simulink model "AXU5EV_Hybrid_ClosedLoop"  (R2026b)
settings: Solver=FixedStepDiscrete  StopTime=6  FixedStep=Ts_Plant
InitFcn:
  | m1a_require_float_init(bdroot);
undefined symbols (not defined in the file): Alignment_Enable, AX01B_Use_C, AX01B_Use_RTL, DiscIntNeverNeededParam, Host_Close_Loop_EN, Host_Id_A, Host_Iq_A, Host_Iq_Test_Mode, Host_Move_Request, Host_PI_Reset_EN, Host_Position_Loop_EN, Host_PWM_EN, Host_Replay_EN, Host_Speed_mmps, Host_Target_mm, Init_Reset, Init_Start, M1A_PWM_Update_Delay_s, PMLSM_Bv_N_per_mps, PMLSM_deadtime_current_eps_A, PMLSM_deadtime_ratio, PMLSM_Fc_N, PMLSM_Kf_peak_N_per_Apeak, PMLSM_Ld_H, PMLSM_Lq_H, PMLSM_M_kg, PMLSM_psi_f_Wb, PMLSM_Rs_ohm, PMLSM_tau_NN_m, PMLSM_theta_offset_rad, PMLSM_Ts_s, PMLSM_v_eps_mps, Simulation_Travel_Fault, Tau_e_mm, theta_align_const, Theta_Offset_Fine, Ts_ACR, Ts_Plant
settings Model: Creator=lww  LastModifiedBy=lww
settings DataIOCC: SaveOutput=off  SaveTime=off

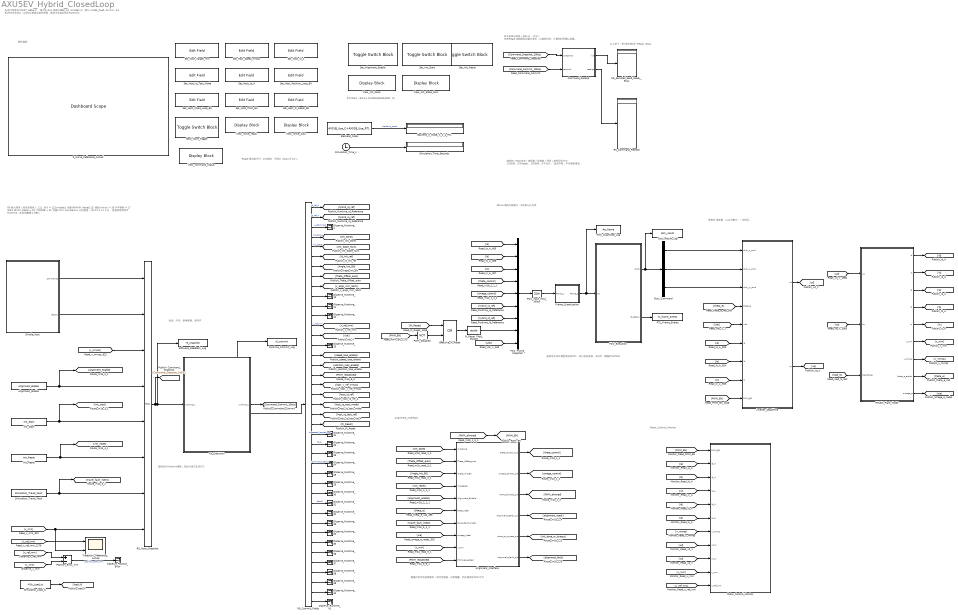
== system AXU5EV_Hybrid_ClosedLoop ==
  note: ​
      | 选择运行Runtime模型，或运行由它生成的C
  note: ​
      | 选择定点FOC模型或实际RTL，执行坐标变换、电流PI、限幅和SVPWM
  note: Alignment_Interface
  note: 根据对齐状态选择固定／实时控制角、应用偏置，并处理实际PWM许可
  note: 轨迹、外环、参考管理、原对齐
  note: Motor_Control_Monitor
  note: 操作面板
  note: 原电机/逆变器，1 µs对象步；一次死区。
  note: 100 µs调用与帧提交；共同50 µs应用
  note: 手动Start；原0.5 A及10000/30000/2000拍
  note: Ready是当拍许可；0时拒绝、不排队（Busy可为0）。
  note: R5 输入顺序（按当前接线）
      | 1:11 命令 → 12:14 replay[速度/PWM/PI_Reset]
      | 15 速度(mm/s) → 16 对齐使能 → 17 Start
      | 18 Init_Reset → 19 行程故障 → 20 位置(mm)
      | Mux/Demux 分组宽度：[11 3 1 1 1 1 1 1]
      | 改变顺序须同步 Runtime，并显式重建 C MEX。
  note: 先运行同目录 START_HERE.m，再点击 Run
      | 参数只编辑 init_AXU5EV.m；默认 model_fixed / 10 mm / 5 s
      | Runtime生成C；Control是独立组件来源，修改不会自动同步Runtime。
  note: 命令采样与回执（100 us，只读）
      | 左侧Ready会随原到位窗口变化；以接收时间、计数和段号确认结果。
  note: 从上到下：R5采样Send / Ready / Busy
  note: 接收秒 / Host状态 / 接受数 / 拒绝数 / 段号 / 接受目标mm
      | 2已接受，3未Ready，5同目标，6不允许；7运动中断，不代表新请求。
  Alignment_Enable : Constant  Value=Alignment_Enable  OutDataTypeStr=double  SampleTime=Ts_ACR
  Alignment_Interface : Subsystem
  Backend_0_Model_1_C_2_RTL : Display
  Backend_Code : Constant  Value=AX01B_Use_C+AX01B_Use_RTL
  Command_Receipt : Subsystem
  Duty_Command : Demux  Outputs=3
  Duty_Result_Log : ToWorkspace  VariableName=duty_result  SaveFormat=Timeseries  SampleTime=Ts_ACR
  Effective_PI_Reset : Logic  Operator=OR  AllPortsSameDT=off  OutDataTypeStr=boolean
  FOC_Execution : Subsystem  Variant=on
  FOC_Frame_Snapshot : Mux  Inputs=9
  FOC_Input_Hold_100us : ZeroOrderHold  SampleTime=Ts_ACR
  FOC_Quantized_Log : ToWorkspace  VariableName=foc_frame  SaveFormat=Timeseries  SampleTime=Ts_ACR
  Frame_Quantization : Subsystem
  Init_Reset : Constant  Value=Init_Reset  SampleTime=Ts_ACR
  Init_Start : Constant  Value=Init_Start  SampleTime=Ts_ACR
  Inverter_DeadTime : Subsystem
  Motor_Control_Monitor : Subsystem
  Observe_Position_Error : Terminator
  Observe_Runtime_{3,10..12,15,24..41} (23 alike) : Terminator
  PI_Reset_Field_Double : DataTypeConversion  OutDataTypeStr=double  SaturateOnIntegerOverflow=off  RndMeth=Floor
  PMLSM_Plant_Model : Subsystem
  PWM_Disabled : Logic  Operator=NOT  AllPortsSameDT=off  OutDataTypeStr=boolean
  Position_Error_mm : Sum  Inputs=+-
  R5_Command_Receipt : Display
  R5_Commit_Fields : Demux  Description=runtime_y（41字段）：1:3 id/iq/v参考；4:12 对齐；13 x_ref_mm；14:23 运行字段；24 接受目标；25 Busy；27 status；31 Ready；32:36 计数/段/中断；37:41 轨迹配置。详见同目录运行说明。  Outputs=41
  R5_Execution : Subsystem  Variant=on
  R5_Input_Snapshot : Mux  Description=runtime_u（20字段）：命令[1:11]，replay[12:14]，v_mmps[15]，Alignment_Enable[16]，Init_Start[17]，Init_Reset[18]，travel_fault[19]，x_mm[20]。保持当前接线顺序，Runtime Demux必须同步。  Inputs=[11 3 1 1 1 1 1 1]
  R5_Sampled_Send_Ready_Busy : Display
  RTL_Frame_Events : ToWorkspace  VariableName=rtl_frame_events  SaveFormat=Timeseries  SampleTime=-1
  Runtime_Commit_Log : ToWorkspace  VariableName=r5_commit  SaveFormat=Timeseries  SampleTime=Ts_ACR
  S_Curve_Reference_Actual : DashboardScope  FontColor=[0.0, 0.0, 0.0]
  Send_Move_Toggle : ToggleSwitchBlock
  Set_Alignment_Enable : ToggleSwitchBlock
  Set_Host_Close_Loop_EN : EditField  ShowInitialText=on  Alignment=Center
  Set_Host_Id_A : EditField  ShowInitialText=on  Alignment=Center
  Set_Host_Iq_A : EditField  ShowInitialText=on  Alignment=Center
  Set_Host_Iq_Test_Mode : EditField  ShowInitialText=on  Alignment=Center
  Set_Host_PI_Reset_EN : EditField  ShowInitialText=on  Alignment=Center
  Set_Host_PWM_EN : EditField  ShowInitialText=on  Alignment=Center
  Set_Host_Position_Loop_EN : EditField  ShowInitialText=on  Alignment=Center
  Set_Host_Speed_mmps : EditField  ShowInitialText=on  Alignment=Center
  Set_Host_Target_mm : EditField  ShowInitialText=on  Alignment=Center
  Set_Init_Reset : ToggleSwitchBlock
  Set_Init_Start : ToggleSwitchBlock
  Simple_Host : Subsystem
  Simulation_Load_N : FromWorkspace  VariableName=M1A_Load_ts  SampleTime=Ts_Plant  Interpolate=off  OutputAfterFinalValue=Holding final value
  Simulation_Time_Seconds : Display
  Simulation_Time_s : Clock
  Simulation_Travel_Fault : Constant  Value=Simulation_Travel_Fault  OutDataTypeStr=double  SampleTime=Ts_ACR
  Software_Feedback_Log : ToWorkspace  VariableName=r5_snapshot  SaveFormat=Timeseries  SampleTime=Ts_ACR
  Trajectory_Reference_Actual : Scope  NumInputPorts=2
      settings: ActiveDisplayYMinimum=0.99182264665726316  ActiveDisplayYMaximum=1.0007838303678565
  View_Init_Done : DisplayBlock  Transparency=1  GridColor=[0.502, 0.502, 0.502]
  View_Init_State_Num : DisplayBlock  Transparency=1  GridColor=[0.502, 0.502, 0.502]
  View_command_status : DisplayBlock  Transparency=1  GridColor=[0.502, 0.502, 0.502]
  View_move_busy : DisplayBlock  Transparency=1  GridColor=[0.502, 0.502, 0.502]
  View_move_ready : DisplayBlock  Transparency=1  GridColor=[0.502, 0.502, 0.502]
  wires:
  [PWM_EN] -> PWM_Disabled/1
  PMLSM_Plant_Model/6(x_mm) -> [x_mm]
  PMLSM_Plant_Model/7(v_mmps) -> [v_mmps]
  PMLSM_Plant_Model/3(ia) -> [ia]
  PMLSM_Plant_Model/4(ib) -> [ib]
  PMLSM_Plant_Model/5(ic) -> [ic]
  PMLSM_Plant_Model/8(theta_e_actual) -> [theta_e]
  PMLSM_Plant_Model/9(omega_e) -> [we]
  PMLSM_Plant_Model/1(id) -> [id]
  PMLSM_Plant_Model/2(iq) -> [iq]
  [load_N] -> PMLSM_Plant_Model/3(load_force)
  [uq] -> PMLSM_Plant_Model/2(vq)
  [ud] -> PMLSM_Plant_Model/1(vd)
  Simulation_Load_N/1 -> [load_N]
  [theta_e] -> Alignment_Interface/6(theta_ideal)
  [we] -> Alignment_Interface/8(omega_ideal)
  Alignment_Interface/1(theta_control_out) -> [theta_control]
  Alignment_Interface/2(omega_control_out) -> [omega_control]
  Alignment_Interface/3(PWM_allowed_out) -> [PWM_allowed]
  [PWM_allowed] -> [PWM_EN]
  Alignment_Interface/4(alignment_ready_out) -> [alignment_ready]
  Alignment_Interface/5(done_or_bypass_out) -> [init_done_or_bypass]
  Alignment_Interface/6(alignment_fault_out) -> [alignment_fault]
  [alignment_enable] -> Alignment_Interface/5(Alignment_Enable)
  [init_reset] -> Alignment_Interface/4(Init_Reset)
  [travel_fault_inject] -> Alignment_Interface/7(travel_fault_inject)
  [PWM_requested] -> Alignment_Interface/10(PWM_requested)
  [Init_Done] -> Alignment_Interface/1(Init_Done)
  [Angle_Init_EN] -> Alignment_Interface/3(Angle_Init_EN)
  [Theta_Offset_auto] -> Alignment_Interface/2(Theta_Offset_auto)
  [x_mm] -> Alignment_Interface/9(x_mm)
  [omega_control] -> FOC_Frame_Snapshot/5
  [theta_control] -> FOC_Frame_Snapshot/4
  [ic] -> FOC_Frame_Snapshot/3
  [ib] -> FOC_Frame_Snapshot/2
  [ia] -> FOC_Frame_Snapshot/1
  [PI_Reset] -> Effective_PI_Reset/1
  PWM_Disabled/1 -> Effective_PI_Reset/2
  FOC_Frame_Snapshot/1 -> FOC_Input_Hold_100us/1
  PI_Reset_Field_Double/1 -> FOC_Frame_Snapshot/8
  Effective_PI_Reset/1 -> PI_Reset_Field_Double/1
  [ic] -> Inverter_DeadTime/8(ic)
  [ib] -> Inverter_DeadTime/7(ib)
  [ia] -> Inverter_DeadTime/6(ia)
  [theta_e] -> Inverter_DeadTime/4(theta_e)
  Inverter_DeadTime/1(vd) -> [ud]
  Inverter_DeadTime/2(vq) -> [uq]
  [PWM_EN] -> Inverter_DeadTime/9(PWM_EN)
  [x_ref_mm] -> Motor_Control_Monitor/11(x_ref_mm)
  [x_mm] -> Motor_Control_Monitor/10(x_mm)
  [uq] -> Motor_Control_Monitor/9(vq_V)
  [ud] -> Motor_Control_Monitor/8(vd_V)
  [v_mmps] -> Motor_Control_Monitor/7(v_mmps)
  [iq] -> Motor_Control_Monitor/6(iq_A)
  [id] -> Motor_Control_Monitor/5(id_A)
  [ic] -> Motor_Control_Monitor/4(ic_A)
  [ib] -> Motor_Control_Monitor/3(ib_A)
  [ia] -> Motor_Control_Monitor/2(ia_A)
  [PWM_EN] -> Motor_Control_Monitor/1(PWM_EN)
  Duty_Command/3 -> Inverter_DeadTime/3(duty_w_cmd)
  Duty_Command/2 -> Inverter_DeadTime/2(duty_v_cmd)
  Duty_Command/1 -> Inverter_DeadTime/1(duty_u_cmd)
  FOC_Execution/1(Out1) -> Duty_Result_Log/1, Duty_Command/1
  FOC_Execution/2(rtl_status) -> RTL_Frame_Events/1
  R5_Commit_Fields/3 -> Observe_Runtime_3/1  "v_ref_mmps"
  R5_Commit_Fields/10 -> Observe_Runtime_10/1
  R5_Commit_Fields/11 -> Observe_Runtime_11/1
  R5_Commit_Fields/12 -> Observe_Runtime_12/1
  R5_Commit_Fields/15 -> Observe_Runtime_15/1
  R5_Commit_Fields/24 -> Observe_Runtime_24/1  "accepted_target_mm"
  R5_Commit_Fields/25 -> Observe_Runtime_25/1  "Busy"
  R5_Commit_Fields/26 -> Observe_Runtime_26/1
  R5_Commit_Fields/27 -> Observe_Runtime_27/1  "command_status"
  R5_Commit_Fields/28 -> Observe_Runtime_28/1
  R5_Commit_Fields/29 -> Observe_Runtime_29/1
  R5_Commit_Fields/30 -> Observe_Runtime_30/1
  R5_Commit_Fields/31 -> Observe_Runtime_31/1  "Ready"
  R5_Commit_Fields/32 -> Observe_Runtime_32/1
  R5_Commit_Fields/33 -> Observe_Runtime_33/1
  R5_Commit_Fields/34 -> Observe_Runtime_34/1
  R5_Commit_Fields/35 -> Observe_Runtime_35/1
  R5_Commit_Fields/36 -> Observe_Runtime_36/1
  R5_Commit_Fields/37 -> Observe_Runtime_37/1
  R5_Commit_Fields/38 -> Observe_Runtime_38/1
  R5_Commit_Fields/39 -> Observe_Runtime_39/1
  R5_Commit_Fields/40 -> Observe_Runtime_40/1
  R5_Commit_Fields/41 -> Observe_Runtime_41/1
  R5_Commit_Fields/4 -> [Init_Done]  "Init_Done"
  R5_Commit_Fields/5 -> [Init_State_Num]  "Init_State"
  R5_Commit_Fields/6 -> [id_init_ref]
  R5_Commit_Fields/7 -> [Angle_Init_EN]
  R5_Commit_Fields/8 -> [Theta_Offset_auto]
  R5_Commit_Fields/9 -> [x_align_mm_latch]
  R5_Commit_Fields/13 -> [x_ref_mm]  "x_ref_mm"
  R5_Commit_Fields/16 -> [speed_loop_enable]
  R5_Commit_Fields/17 -> [position_loop_enable]
  R5_Commit_Fields/20 -> [host_id_ref]
  R5_Commit_Fields/21 -> [host_iq_test_mode]
  R5_Commit_Fields/22 -> [host_iq_test_ref]
  R5_Commit_Fields/19 -> [host_v_ref_mmps]
  R5_Commit_Fields/18 -> [PWM_requested]
  R5_Commit_Fields/23 -> [PI_Reset]
  FOC_Input_Hold_100us/1 -> Frame_Quantization/1(frame_u)
  Frame_Quantization/1(frame_q) -> FOC_Quantized_Log/1, FOC_Execution/1(In1)
  Alignment_Enable/1 -> [alignment_enable], R5_Input_Snapshot/4
  Init_Start/1 -> [init_start], R5_Input_Snapshot/5
  Init_Reset/1 -> [init_reset], R5_Input_Snapshot/6
  Simulation_Travel_Fault/1 -> [travel_fault_inject], R5_Input_Snapshot/7
  [x_ref_mm] -> Trajectory_Reference_Actual/1
  [x_mm] -> Trajectory_Reference_Actual/2, R5_Input_Snapshot/8
  Simple_Host/1(commands) -> R5_Input_Snapshot/1
  [v_mmps] -> R5_Input_Snapshot/3
  [hybrid_iq_ref] -> FOC_Frame_Snapshot/6
  [hybrid_id_ref] -> FOC_Frame_Snapshot/7
  R5_Commit_Fields/1 -> [hybrid_id_ref]  "id_ref_A"
  R5_Commit_Fields/2 -> [hybrid_iq_ref]  "iq_ref_A"
  R5_Commit_Fields/14 -> [Udc]
  [Udc] -> FOC_Frame_Snapshot/9
  Simple_Host/2(replay) -> R5_Input_Snapshot/2
  [Udc] -> Inverter_DeadTime/5(vdc)
  Position_Error_mm/1 -> Observe_Position_Error/1  "position_error_mm"
  [x_mm] -> Position_Error_mm/2
  [x_ref_mm] -> Position_Error_mm/1
  Simulation_Time_s/1 -> Simulation_Time_Seconds/1
  Backend_Code/1 -> Backend_0_Model_1_C_2_RTL/1  "backend_code"
  Command_Receipt/2(receipt) -> R5_Command_Receipt/1
  Command_Receipt/1(live) -> R5_Sampled_Send_Ready_Busy/1
  [Command_Commit_100us] -> Command_Receipt/2(commit)
  [Command_Snapshot_100us] -> Command_Receipt/1(snapshot)
  R5_Input_Snapshot/1 -> R5_Execution/1(runtime_u), Software_Feedback_Log/1, [Command_Snapshot_100us]
  R5_Execution/1(runtime_y) -> [Command_Commit_100us], Runtime_Commit_Log/1, R5_Commit_Fields/1

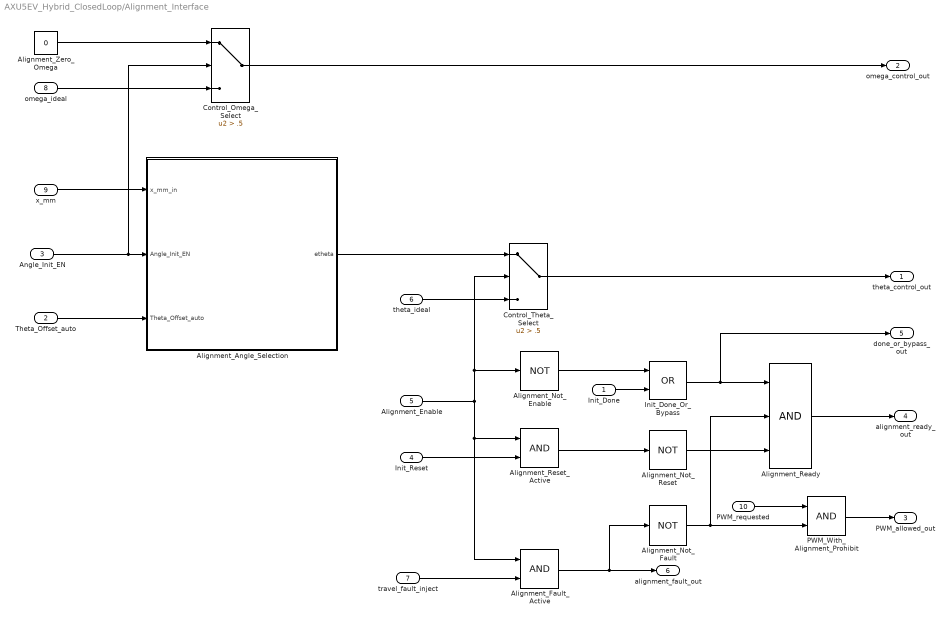
== system AXU5EV_Hybrid_ClosedLoop/Alignment_Interface ==
  Init_Done : Inport
  Theta_Offset_auto : Inport  Port=2
  Angle_Init_EN : Inport  Port=3
  Init_Reset : Inport  Port=4
  Alignment_Enable : Inport  Port=5
  theta_ideal : Inport  Port=6
  travel_fault_inject : Inport  Port=7
  omega_ideal : Inport  Port=8
  x_mm : Inport  Port=9
  PWM_requested : Inport  Port=10
  Alignment_Angle_Selection : Subsystem
  Alignment_Fault_Active : Logic  AllPortsSameDT=off  OutDataTypeStr=boolean
  Alignment_Not_Enable : Logic  Operator=NOT  AllPortsSameDT=off  OutDataTypeStr=boolean
  Alignment_Not_Fault : Logic  Operator=NOT  AllPortsSameDT=off  OutDataTypeStr=boolean
  Alignment_Not_Reset : Logic  Operator=NOT  AllPortsSameDT=off  OutDataTypeStr=boolean
  Alignment_Ready : Logic  Inputs=3  AllPortsSameDT=off  OutDataTypeStr=boolean
  Alignment_Reset_Active : Logic  AllPortsSameDT=off  OutDataTypeStr=boolean
  Alignment_Zero_Omega : Constant  Value=0
  Control_Omega_Select : Switch  Criteria=u2 > Threshold  Threshold=.5
  Control_Theta_Select : Switch  Criteria=u2 > Threshold  Threshold=.5
  Init_Done_Or_Bypass : Logic  Operator=OR  AllPortsSameDT=off  OutDataTypeStr=boolean
  PWM_With_Alignment_Prohibit : Logic  AllPortsSameDT=off  OutDataTypeStr=boolean
  theta_control_out : Outport
  omega_control_out : Outport  Port=2
  PWM_allowed_out : Outport  Port=3
  alignment_ready_out : Outport  Port=4
  done_or_bypass_out : Outport  Port=5
  alignment_fault_out : Outport  Port=6
  wires:
  Alignment_Zero_Omega/1 -> Control_Omega_Select/1
  travel_fault_inject/1 -> Alignment_Fault_Active/2
  x_mm/1 -> Alignment_Angle_Selection/1(x_mm_in)
  Alignment_Enable/1 -> Alignment_Fault_Active/1, Alignment_Reset_Active/1, Alignment_Not_Enable/1, Control_Theta_Select/2
  PWM_requested/1 -> PWM_With_Alignment_Prohibit/1
  omega_ideal/1 -> Control_Omega_Select/3
  theta_ideal/1 -> Control_Theta_Select/3
  Angle_Init_EN/1 -> Control_Omega_Select/2, Alignment_Angle_Selection/2(Angle_Init_EN)
  Init_Reset/1 -> Alignment_Reset_Active/2
  Theta_Offset_auto/1 -> Alignment_Angle_Selection/3(Theta_Offset_auto)
  Control_Omega_Select/1 -> omega_control_out/1
  Alignment_Angle_Selection/1(etheta) -> Control_Theta_Select/1
  PWM_With_Alignment_Prohibit/1 -> PWM_allowed_out/1
  Init_Done_Or_Bypass/1 -> done_or_bypass_out/1, Alignment_Ready/1
  Control_Theta_Select/1 -> theta_control_out/1
  Alignment_Fault_Active/1 -> Alignment_Not_Fault/1, alignment_fault_out/1
  Alignment_Not_Enable/1 -> Init_Done_Or_Bypass/1
  Alignment_Not_Reset/1 -> Alignment_Ready/3
  Alignment_Reset_Active/1 -> Alignment_Not_Reset/1
  Alignment_Not_Fault/1 -> Alignment_Ready/2, PWM_With_Alignment_Prohibit/2
  Alignment_Ready/1 -> alignment_ready_out/1
  Init_Done/1 -> Init_Done_Or_Bypass/2

== system AXU5EV_Hybrid_ClosedLoop/Command_Receipt ==
  snapshot : Inport
  commit : Inport  Port=2
  Receipt_Fields : MATLAB Function  TreatAsAtomicUnit=on
  Snapshot_100us : ZeroOrderHold  SampleTime=Ts_ACR
  live : Outport
  receipt : Outport  Port=2
  wires:
  Snapshot_100us/1 -> Receipt_Fields/1(snapshot)
  snapshot/1 -> Snapshot_100us/1
  commit/1 -> Receipt_Fields/2(commit)
  Receipt_Fields/1(live) -> live/1
  Receipt_Fields/2(receipt) -> receipt/1

== system AXU5EV_Hybrid_ClosedLoop/FOC_Execution ==
  note: 1) Add Subsystem or Model blocks as valid variant choices.
      | 2) You cannot connect blocks at this level. At simulation, connectivity is automatically
      | determined, based on the active variant and port name matching.
  In1 : Inport
  Fixed_Reference : Subsystem  VariantControl=AX01B_Use_RTL == 0
  P3_RTL : Subsystem  VariantControl=AX01B_Use_RTL == 1
  Out1 : Outport
  rtl_status : Outport  Port=2

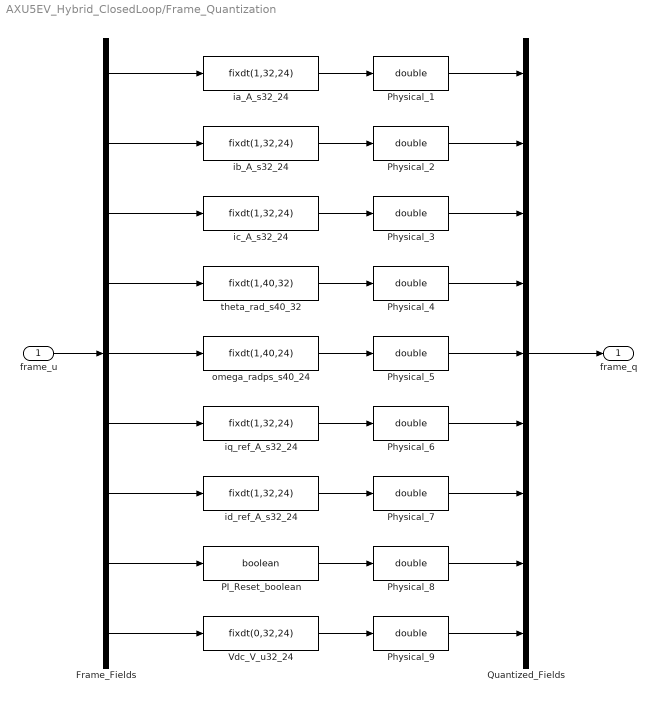
== system AXU5EV_Hybrid_ClosedLoop/Frame_Quantization ==
  frame_u : Inport
  Frame_Fields : Demux  Outputs=9
  PI_Reset_boolean : DataTypeConversion  OutDataTypeStr=boolean  RndMeth=Convergent
  Physical_{1..9} (9 alike) : DataTypeConversion  OutDataTypeStr=double  SaturateOnIntegerOverflow=off  RndMeth=Floor
  Quantized_Fields : Mux  Inputs=9
  Vdc_V_u32_24 : DataTypeConversion  OutDataTypeStr=fixdt(0,32,24)  RndMeth=Convergent
  ia_A_s32_24 : DataTypeConversion  OutDataTypeStr=fixdt(1,32,24)  RndMeth=Convergent
  ib_A_s32_24 : DataTypeConversion  OutDataTypeStr=fixdt(1,32,24)  RndMeth=Convergent
  ic_A_s32_24 : DataTypeConversion  OutDataTypeStr=fixdt(1,32,24)  RndMeth=Convergent
  id_ref_A_s32_24 : DataTypeConversion  OutDataTypeStr=fixdt(1,32,24)  RndMeth=Convergent
  iq_ref_A_s32_24 : DataTypeConversion  OutDataTypeStr=fixdt(1,32,24)  RndMeth=Convergent
  omega_radps_s40_24 : DataTypeConversion  OutDataTypeStr=fixdt(1,40,24)  RndMeth=Convergent
  theta_rad_s40_32 : DataTypeConversion  OutDataTypeStr=fixdt(1,40,32)  RndMeth=Convergent
  frame_q : Outport
  wires:
  Quantized_Fields/1 -> frame_q/1
  Physical_9/1 -> Quantized_Fields/9
  Vdc_V_u32_24/1 -> Physical_9/1
  Frame_Fields/9 -> Vdc_V_u32_24/1
  Physical_8/1 -> Quantized_Fields/8
  PI_Reset_boolean/1 -> Physical_8/1
  Frame_Fields/8 -> PI_Reset_boolean/1
  Physical_7/1 -> Quantized_Fields/7
  id_ref_A_s32_24/1 -> Physical_7/1
  Frame_Fields/7 -> id_ref_A_s32_24/1
  Physical_6/1 -> Quantized_Fields/6
  iq_ref_A_s32_24/1 -> Physical_6/1
  Frame_Fields/6 -> iq_ref_A_s32_24/1
  Physical_5/1 -> Quantized_Fields/5
  omega_radps_s40_24/1 -> Physical_5/1
  Frame_Fields/5 -> omega_radps_s40_24/1
  Physical_4/1 -> Quantized_Fields/4
  theta_rad_s40_32/1 -> Physical_4/1
  Frame_Fields/4 -> theta_rad_s40_32/1
  Physical_3/1 -> Quantized_Fields/3
  ic_A_s32_24/1 -> Physical_3/1
  Frame_Fields/3 -> ic_A_s32_24/1
  Physical_2/1 -> Quantized_Fields/2
  ib_A_s32_24/1 -> Physical_2/1
  Frame_Fields/2 -> ib_A_s32_24/1
  Physical_1/1 -> Quantized_Fields/1
  ia_A_s32_24/1 -> Physical_1/1
  Frame_Fields/1 -> ia_A_s32_24/1
  frame_u/1 -> Frame_Fields/1

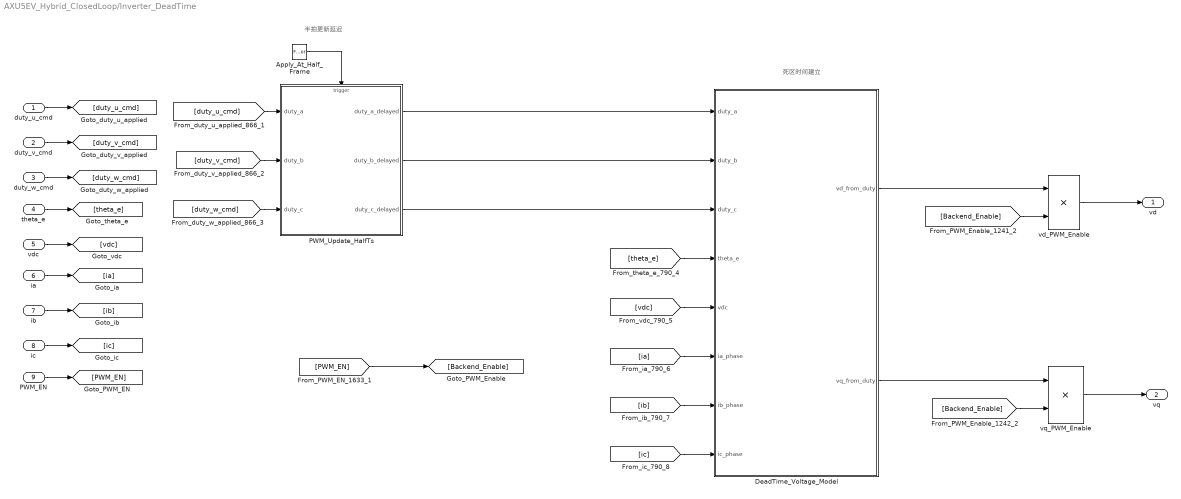
== system AXU5EV_Hybrid_ClosedLoop/Inverter_DeadTime ==
  note: 死区时间建立
  note: 半拍更新延迟
  duty_u_cmd : Inport
  duty_v_cmd : Inport  Port=2
  duty_w_cmd : Inport  Port=3
  theta_e : Inport  Port=4
  vdc : Inport  Port=5
  ia : Inport  Port=6
  ib : Inport  Port=7
  ic : Inport  Port=8
  PWM_EN : Inport  Port=9
  Apply_At_Half_Frame : FunctionCallGenerator  SampleTime=[Ts_ACR M1A_PWM_Update_Delay_s]
  DeadTime_Voltage_Model : Subsystem
  PWM_Update_HalfTs : Subsystem
  vd_PWM_Enable : Product  Inputs=**
  vq_PWM_Enable : Product  Inputs=**
  vd : Outport
  vq : Outport  Port=2
  wires:
  [PWM_EN] -> [Backend_Enable]
  [ic] -> DeadTime_Voltage_Model/8(ic_phase)
  [ib] -> DeadTime_Voltage_Model/7(ib_phase)
  [ia] -> DeadTime_Voltage_Model/6(ia_phase)
  [vdc] -> DeadTime_Voltage_Model/5(vdc)
  [theta_e] -> DeadTime_Voltage_Model/4(theta_e)
  [duty_w_cmd] -> PWM_Update_HalfTs/3(duty_c)
  [duty_v_cmd] -> PWM_Update_HalfTs/2(duty_b)
  [duty_u_cmd] -> PWM_Update_HalfTs/1(duty_a)
  PWM_EN/1 -> [PWM_EN]
  PWM_Update_HalfTs/3(duty_c_delayed) -> DeadTime_Voltage_Model/3(duty_c)
  PWM_Update_HalfTs/2(duty_b_delayed) -> DeadTime_Voltage_Model/2(duty_b)
  PWM_Update_HalfTs/1(duty_a_delayed) -> DeadTime_Voltage_Model/1(duty_a)
  ic/1 -> [ic]
  ib/1 -> [ib]
  ia/1 -> [ia]
  vdc/1 -> [vdc]
  theta_e/1 -> [theta_e]
  duty_u_cmd/1 -> [duty_u_cmd]
  duty_v_cmd/1 -> [duty_v_cmd]
  duty_w_cmd/1 -> [duty_w_cmd]
  [Backend_Enable] -> vd_PWM_Enable/2
  [Backend_Enable] -> vq_PWM_Enable/2
  DeadTime_Voltage_Model/1(vd_from_duty) -> vd_PWM_Enable/1
  DeadTime_Voltage_Model/2(vq_from_duty) -> vq_PWM_Enable/1
  vd_PWM_Enable/1 -> vd/1
  vq_PWM_Enable/1 -> vq/1
  Apply_At_Half_Frame/1 -> PWM_Update_HalfTs/Trigger

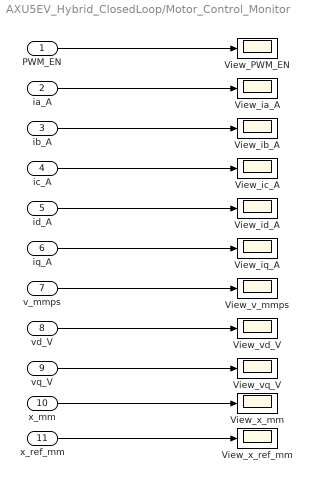
== system AXU5EV_Hybrid_ClosedLoop/Motor_Control_Monitor ==
  PWM_EN : Inport
  ia_A : Inport  Port=2
  ib_A : Inport  Port=3
  ic_A : Inport  Port=4
  id_A : Inport  Port=5
  iq_A : Inport  Port=6
  v_mmps : Inport  Port=7
  vd_V : Inport  Port=8
  vq_V : Inport  Port=9
  x_mm : Inport  Port=10
  x_ref_mm : Inport  Port=11
  View_PWM_EN : Scope
  View_ia_A : Scope
  View_ib_A : Scope
  View_ic_A : Scope
  View_id_A : Scope
  View_iq_A : Scope
  View_v_mmps : Scope
  View_vd_V : Scope
  View_vq_V : Scope
  View_x_mm : Scope
  View_x_ref_mm : Scope
  wires:
  PWM_EN/1 -> View_PWM_EN/1
  ia_A/1 -> View_ia_A/1
  ib_A/1 -> View_ib_A/1
  ic_A/1 -> View_ic_A/1
  id_A/1 -> View_id_A/1
  iq_A/1 -> View_iq_A/1
  v_mmps/1 -> View_v_mmps/1
  vd_V/1 -> View_vd_V/1
  vq_V/1 -> View_vq_V/1
  x_mm/1 -> View_x_mm/1
  x_ref_mm/1 -> View_x_ref_mm/1

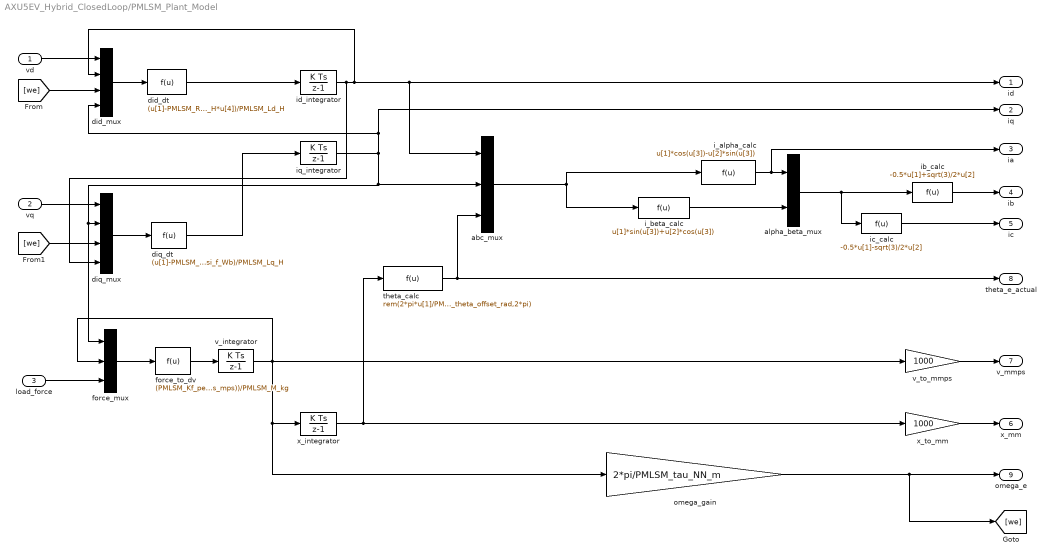
== system AXU5EV_Hybrid_ClosedLoop/PMLSM_Plant_Model ==
  vd : Inport
  vq : Inport  Port=2
  load_force : Inport  Port=3
  abc_mux : Mux  Inputs=3
  alpha_beta_mux : Mux  Inputs=2
  did_dt : Fcn  Expr=(u[1]-PMLSM_Rs_ohm*u[2]+u[3]*PMLSM_Lq_H*u[4])/PMLSM_Ld_H
  did_mux : Mux
  diq_dt : Fcn  Expr=(u[1]-PMLSM_Rs_ohm*u[2]-u[3]*PMLSM_Ld_H*u[4]-u[3]*PMLSM_psi_f_Wb)/PMLSM_Lq_H
  diq_mux : Mux
  force_mux : Mux  Inputs=3
  force_to_dv : Fcn  Expr=(PMLSM_Kf_peak_N_per_Apeak*u[1]-u[3]-PMLSM_Bv_N_per_mps*u[2]-PMLSM_Fc_N*tanh(u[2]/PMLSM_v_eps_mps))/PMLSM_M_kg
  i_alpha_calc : Fcn  Expr=u[1]*cos(u[3])-u[2]*sin(u[3])
  i_beta_calc : Fcn  Expr=u[1]*sin(u[3])+u[2]*cos(u[3])
  ib_calc : Fcn  Expr=-0.5*u[1]+sqrt(3)/2*u[2]
  ic_calc : Fcn  Expr=-0.5*u[1]-sqrt(3)/2*u[2]
  id_integrator : DiscreteIntegrator  gainval=1  SampleTime=PMLSM_Ts_s  ICPrevOutput=DiscIntNeverNeededParam  ICPrevScaledInput=DiscIntNeverNeededParam
  iq_integrator : DiscreteIntegrator  gainval=1  SampleTime=PMLSM_Ts_s  ICPrevOutput=DiscIntNeverNeededParam  ICPrevScaledInput=DiscIntNeverNeededParam
  omega_gain : Gain  Gain=2*pi/PMLSM_tau_NN_m
  theta_calc : Fcn  Expr=rem(2*pi*u[1]/PMLSM_tau_NN_m+PMLSM_theta_offset_rad,2*pi)
  v_integrator : DiscreteIntegrator  gainval=1  SampleTime=PMLSM_Ts_s  ICPrevOutput=DiscIntNeverNeededParam  ICPrevScaledInput=DiscIntNeverNeededParam
  v_to_mmps : Gain  Gain=1000
  x_integrator : DiscreteIntegrator  gainval=1  SampleTime=PMLSM_Ts_s  ICPrevOutput=DiscIntNeverNeededParam  ICPrevScaledInput=DiscIntNeverNeededParam
  x_to_mm : Gain  Gain=1000
  id : Outport
  iq : Outport  Port=2
  ia : Outport  Port=3
  ib : Outport  Port=4
  ic : Outport  Port=5
  x_mm : Outport  Port=6
  v_mmps : Outport  Port=7
  theta_e_actual : Outport  Port=8
  omega_e : Outport  Port=9
  wires:
  ic_calc/1 -> ic/1
  ib_calc/1 -> ib/1
  alpha_beta_mux/1 -> ic_calc/1, ib_calc/1
  i_beta_calc/1 -> alpha_beta_mux/2
  i_alpha_calc/1 -> alpha_beta_mux/1, ia/1
  force_to_dv/1 -> v_integrator/1
  force_mux/1 -> force_to_dv/1
  load_force/1 -> force_mux/3
  diq_dt/1 -> iq_integrator/1
  diq_mux/1 -> diq_dt/1
  vq/1 -> diq_mux/1
  did_dt/1 -> id_integrator/1
  did_mux/1 -> did_dt/1
  vd/1 -> did_mux/1
  x_to_mm/1 -> x_mm/1
  v_to_mmps/1 -> v_mmps/1
  theta_calc/1 -> theta_e_actual/1, abc_mux/3
  omega_gain/1 -> [we], omega_e/1
  id_integrator/1 -> id/1, abc_mux/1, did_mux/2, diq_mux/4
  iq_integrator/1 -> abc_mux/2, force_mux/1, diq_mux/2, iq/1, did_mux/4
  v_integrator/1 -> omega_gain/1, x_integrator/1, v_to_mmps/1, force_mux/2
  x_integrator/1 -> theta_calc/1, x_to_mm/1
  abc_mux/1 -> i_alpha_calc/1, i_beta_calc/1
  [we] -> did_mux/3
  [we] -> diq_mux/3

== system AXU5EV_Hybrid_ClosedLoop/R5_Execution ==
  note: 选择运行Runtime模型，或运行由它生成的C
  note: 1) Add Subsystem or Model blocks as valid variant choices.
      | 2) You cannot connect blocks at this level. At simulation, connectivity is automatically
      | determined, based on the active variant and port name matching.
  runtime_u : Inport
  Generated_C : Subsystem  VariantControl=AX01B_Use_C == 1
  Model_Runtime : ModelReference  ModelNameDialog=AXU5EV_R5_Runtime  SimulationMode=Normal  VariantControl=AX01B_Use_C == 0  ModelReferenceVersion=1.49
  runtime_y : Outport

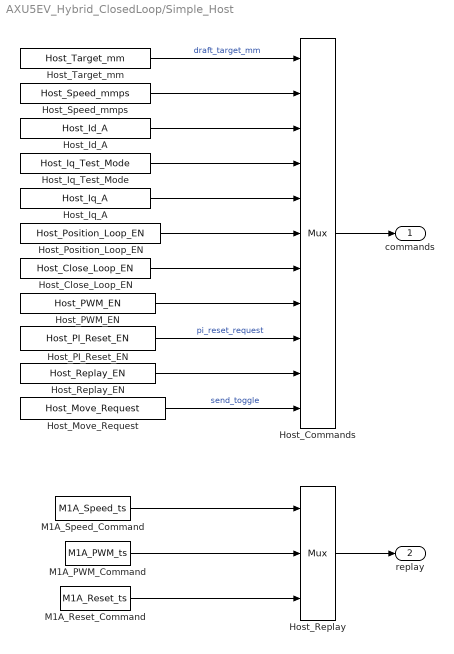
== system AXU5EV_Hybrid_ClosedLoop/Simple_Host ==
  Host_Close_Loop_EN : Constant  Value=Host_Close_Loop_EN  SampleTime=Ts_ACR
  Host_Commands : Mux  Inputs=11
  Host_Id_A : Constant  Value=Host_Id_A  SampleTime=Ts_ACR
  Host_Iq_A : Constant  Value=Host_Iq_A  SampleTime=Ts_ACR
  Host_Iq_Test_Mode : Constant  Value=Host_Iq_Test_Mode  SampleTime=Ts_ACR
  Host_Move_Request : Constant  Value=Host_Move_Request  SampleTime=Ts_ACR
  Host_PI_Reset_EN : Constant  Value=Host_PI_Reset_EN  SampleTime=Ts_ACR
  Host_PWM_EN : Constant  Value=Host_PWM_EN  SampleTime=Ts_ACR
  Host_Position_Loop_EN : Constant  Value=Host_Position_Loop_EN  SampleTime=Ts_ACR
  Host_Replay : Mux  Inputs=3
  Host_Replay_EN : Constant  Value=Host_Replay_EN  SampleTime=Ts_ACR
  Host_Speed_mmps : Constant  Value=Host_Speed_mmps  SampleTime=Ts_ACR
  Host_Target_mm : Constant  Value=Host_Target_mm  SampleTime=Ts_ACR
  M1A_PWM_Command : FromWorkspace  VariableName=M1A_PWM_ts  SampleTime=Ts_Plant  Interpolate=off  OutputAfterFinalValue=Holding final value
  M1A_Reset_Command : FromWorkspace  VariableName=M1A_Reset_ts  SampleTime=Ts_Plant  Interpolate=off  OutputAfterFinalValue=Holding final value
  M1A_Speed_Command : FromWorkspace  VariableName=M1A_Speed_ts  SampleTime=Ts_Plant  Interpolate=off  OutputAfterFinalValue=Holding final value
  commands : Outport
  replay : Outport  Port=2
  wires:
  Host_Target_mm/1 -> Host_Commands/1  "draft_target_mm"
  Host_Speed_mmps/1 -> Host_Commands/2
  Host_Id_A/1 -> Host_Commands/3
  Host_PWM_EN/1 -> Host_Commands/8
  M1A_Speed_Command/1 -> Host_Replay/1
  Host_Iq_Test_Mode/1 -> Host_Commands/4
  Host_Position_Loop_EN/1 -> Host_Commands/6
  M1A_Reset_Command/1 -> Host_Replay/3
  Host_Iq_A/1 -> Host_Commands/5
  Host_Close_Loop_EN/1 -> Host_Commands/7
  Host_PI_Reset_EN/1 -> Host_Commands/9  "pi_reset_request"
  Host_Replay_EN/1 -> Host_Commands/10
  Host_Move_Request/1 -> Host_Commands/11  "send_toggle"
  M1A_PWM_Command/1 -> Host_Replay/2
  Host_Replay/1 -> replay/1
  Host_Commands/1 -> commands/1

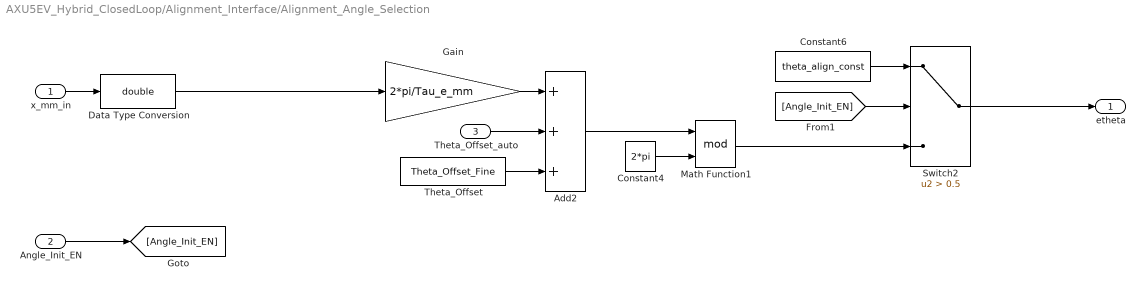
== system AXU5EV_Hybrid_ClosedLoop/Alignment_Interface/Alignment_Angle_Selection ==
  x_mm_in : Inport
  Angle_Init_EN : Inport  Port=2
  Theta_Offset_auto : Inport  Port=3
  Add2 : Sum  Inputs=+++
  Constant4 : Constant  Value=2*pi
  Constant6 : Constant  Value=theta_align_const
  Data Type Conversion : DataTypeConversion  OutDataTypeStr=double  SaturateOnIntegerOverflow=off  RndMeth=Floor
  Gain : Gain  Gain=2*pi/Tau_e_mm
  Math Function1 : Math  Operator=mod
  Switch2 : Switch  Criteria=u2 > Threshold  Threshold=0.5  SaturateOnIntegerOverflow=off  InputSameDT=off
  Theta_Offset : Constant  Value=Theta_Offset_Fine
  etheta : Outport
  wires:
  Gain/1 -> Add2/1
  Theta_Offset_auto/1 -> Add2/2
  Theta_Offset/1 -> Add2/3
  x_mm_in/1 -> Data Type Conversion/1
  Data Type Conversion/1 -> Gain/1
  Angle_Init_EN/1 -> [Angle_Init_EN]
  Add2/1 -> Math Function1/1
  Constant4/1 -> Math Function1/2
  Constant6/1 -> Switch2/1
  [Angle_Init_EN] -> Switch2/2
  Math Function1/1 -> Switch2/3
  Switch2/1 -> etheta/1

== system AXU5EV_Hybrid_ClosedLoop/FOC_Execution/Fixed_Reference ==
  In1 : Inport
  Accepted_Fixed_FOC : Subsystem  VariantControl=FOC_Impl_Select == 1
  Duty_Vector : Mux  Inputs=3
  FOC_Fields : Demux  Outputs=9
  Not_RTL_Status : Constant  Value=zeros(1,4)
  Out1 : Outport
  rtl_status : Outport  Port=2
  wires:
  Not_RTL_Status/1 -> rtl_status/1
  In1/1 -> FOC_Fields/1
  FOC_Fields/1 -> Accepted_Fixed_FOC/1(ia)
  FOC_Fields/2 -> Accepted_Fixed_FOC/2(ib)
  FOC_Fields/3 -> Accepted_Fixed_FOC/3(ic)
  FOC_Fields/4 -> Accepted_Fixed_FOC/4(theta_e)
  FOC_Fields/5 -> Accepted_Fixed_FOC/5(omega_e)
  FOC_Fields/6 -> Accepted_Fixed_FOC/6(iq_ref)
  FOC_Fields/7 -> Accepted_Fixed_FOC/7(id_ref)
  FOC_Fields/8 -> Accepted_Fixed_FOC/8(PI_Reset_EN)
  FOC_Fields/9 -> Accepted_Fixed_FOC/9(Vdc_V)
  Accepted_Fixed_FOC/1(duty_u_cmd) -> Duty_Vector/1
  Accepted_Fixed_FOC/2(duty_v_cmd) -> Duty_Vector/2
  Accepted_Fixed_FOC/3(duty_w_cmd) -> Duty_Vector/3
  Duty_Vector/1 -> Out1/1

== system AXU5EV_Hybrid_ClosedLoop/FOC_Execution/P3_RTL ==
  In1 : Inport
  Actual_P3_XSI : S-Function  FunctionName=ax01b_foc_xsi_sfun  Parameters=AX01B_XSI_Work, AX01B_Vivado_Root  SFunctionDeploymentMode=off  EnableBusSupport=off
  Out1 : Outport
  rtl_status : Outport  Port=2
  wires:
  Actual_P3_XSI/1 -> Out1/1
  In1/1 -> Actual_P3_XSI/1
  Actual_P3_XSI/2 -> rtl_status/1

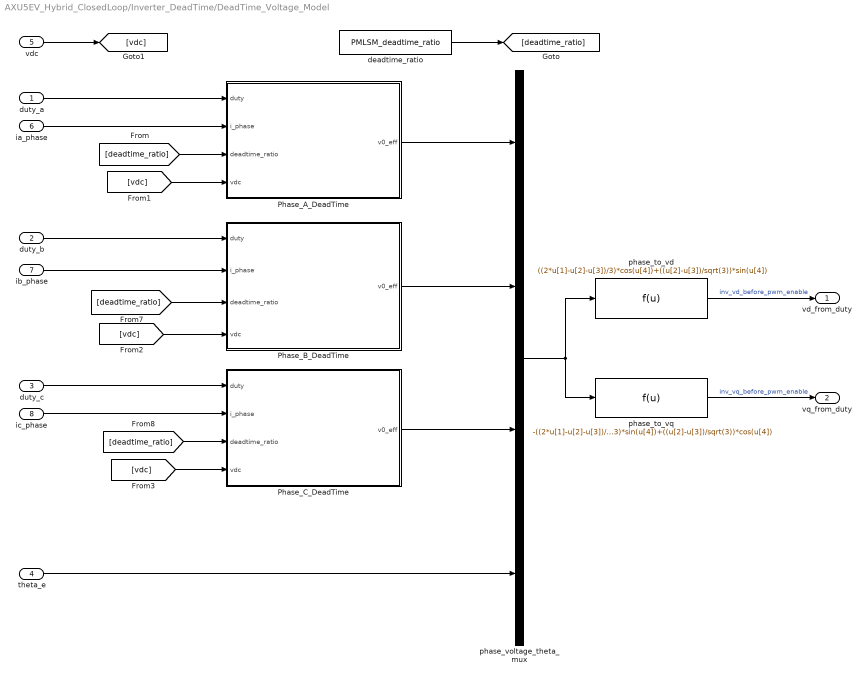
== system AXU5EV_Hybrid_ClosedLoop/Inverter_DeadTime/DeadTime_Voltage_Model ==
  duty_a : Inport
  duty_b : Inport  Port=2
  duty_c : Inport  Port=3
  theta_e : Inport  Port=4
  vdc : Inport  Port=5
  ia_phase : Inport  Port=6
  ib_phase : Inport  Port=7
  ic_phase : Inport  Port=8
  Phase_A_DeadTime : Subsystem
  Phase_B_DeadTime : Subsystem
  Phase_C_DeadTime : Subsystem
  deadtime_ratio : Constant  Value=PMLSM_deadtime_ratio
  phase_to_vd : Fcn  Expr=((2*u[1]-u[2]-u[3])/3)*cos(u[4])+((u[2]-u[3])/sqrt(3))*sin(u[4])
  phase_to_vq : Fcn  Expr=-((2*u[1]-u[2]-u[3])/3)*sin(u[4])+((u[2]-u[3])/sqrt(3))*cos(u[4])
  phase_voltage_theta_mux : Mux
  vd_from_duty : Outport
  vq_from_duty : Outport  Port=2
  wires:
  [deadtime_ratio] -> Phase_C_DeadTime/3(deadtime_ratio)
  [deadtime_ratio] -> Phase_B_DeadTime/3(deadtime_ratio)
  [deadtime_ratio] -> Phase_A_DeadTime/3(deadtime_ratio)
  [vdc] -> Phase_C_DeadTime/4(vdc)
  [vdc] -> Phase_B_DeadTime/4(vdc)
  [vdc] -> Phase_A_DeadTime/4(vdc)
  vdc/1 -> [vdc]
  theta_e/1 -> phase_voltage_theta_mux/4
  Phase_C_DeadTime/1(v0_eff) -> phase_voltage_theta_mux/3
  Phase_B_DeadTime/1(v0_eff) -> phase_voltage_theta_mux/2
  Phase_A_DeadTime/1(v0_eff) -> phase_voltage_theta_mux/1
  ic_phase/1 -> Phase_C_DeadTime/2(i_phase)
  duty_c/1 -> Phase_C_DeadTime/1(duty)
  ib_phase/1 -> Phase_B_DeadTime/2(i_phase)
  duty_b/1 -> Phase_B_DeadTime/1(duty)
  ia_phase/1 -> Phase_A_DeadTime/2(i_phase)
  duty_a/1 -> Phase_A_DeadTime/1(duty)
  deadtime_ratio/1 -> [deadtime_ratio]
  phase_to_vq/1 -> vq_from_duty/1  "inv_vq_before_pwm_enable"
  phase_to_vd/1 -> vd_from_duty/1  "inv_vd_before_pwm_enable"
  phase_voltage_theta_mux/1 -> phase_to_vd/1, phase_to_vq/1

== system AXU5EV_Hybrid_ClosedLoop/Inverter_DeadTime/PWM_Update_HalfTs ==
  duty_a : Inport
  duty_b : Inport  Port=2
  duty_c : Inport  Port=3
  Apply_50us : TriggerPort  TriggerType=function-call  VariantControl=(inherit)  PortDimensions=1
  duty_a_delayed : Outport  InitialOutput=0.5
  duty_b_delayed : Outport  Port=2  InitialOutput=0.5
  duty_c_delayed : Outport  Port=3  InitialOutput=0.5
  wires:
  duty_c/1 -> duty_c_delayed/1
  duty_b/1 -> duty_b_delayed/1
  duty_a/1 -> duty_a_delayed/1

== system AXU5EV_Hybrid_ClosedLoop/R5_Execution/Generated_C ==
  runtime_u : Inport
  Generated_Runtime_Step : S-Function  FunctionName=ax01b_r5_sfun  SFunctionDeploymentMode=off  EnableBusSupport=off
  runtime_y : Outport
  wires:
  Generated_Runtime_Step/1 -> runtime_y/1
  runtime_u/1 -> Generated_Runtime_Step/1

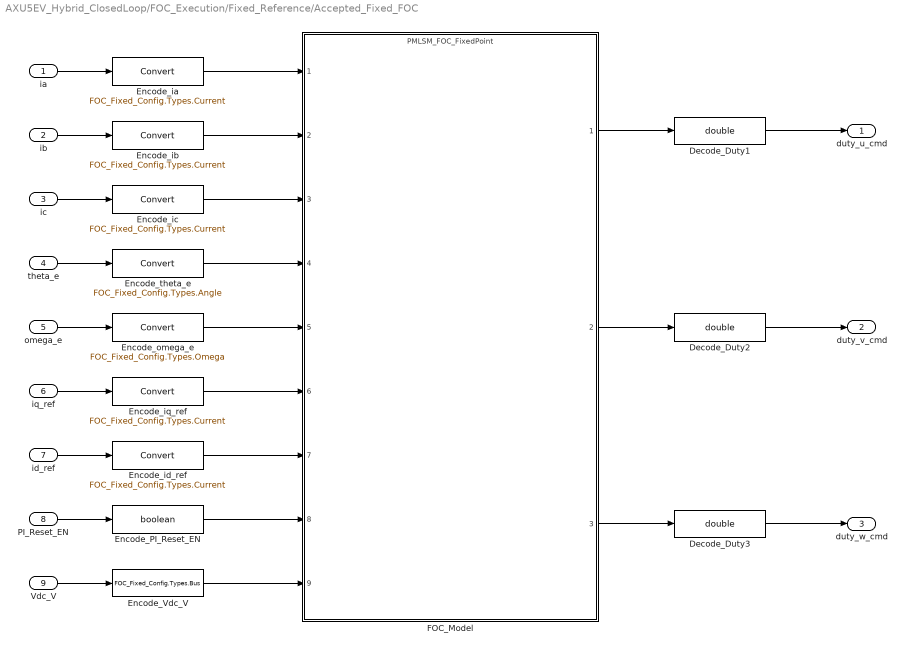
== system AXU5EV_Hybrid_ClosedLoop/FOC_Execution/Fixed_Reference/Accepted_Fixed_FOC ==
  ia : Inport
  ib : Inport  Port=2
  ic : Inport  Port=3
  theta_e : Inport  Port=4
  omega_e : Inport  Port=5
  iq_ref : Inport  Port=6
  id_ref : Inport  Port=7
  PI_Reset_EN : Inport  Port=8
  Vdc_V : Inport  Port=9
  Decode_Duty1 : DataTypeConversion  OutDataTypeStr=double
  Decode_Duty2 : DataTypeConversion  OutDataTypeStr=double
  Decode_Duty3 : DataTypeConversion  OutDataTypeStr=double
  Encode_PI_Reset_EN : DataTypeConversion  OutDataTypeStr=boolean  RndMeth=Convergent
  Encode_Vdc_V : DataTypeConversion  OutDataTypeStr=FOC_Fixed_Config.Types.Bus  RndMeth=Convergent
  Encode_ia : DataTypeConversion  OutDataTypeStr=FOC_Fixed_Config.Types.Current  RndMeth=Convergent
  Encode_ib : DataTypeConversion  OutDataTypeStr=FOC_Fixed_Config.Types.Current  RndMeth=Convergent
  Encode_ic : DataTypeConversion  OutDataTypeStr=FOC_Fixed_Config.Types.Current  RndMeth=Convergent
  Encode_id_ref : DataTypeConversion  OutDataTypeStr=FOC_Fixed_Config.Types.Current  RndMeth=Convergent
  Encode_iq_ref : DataTypeConversion  OutDataTypeStr=FOC_Fixed_Config.Types.Current  RndMeth=Convergent
  Encode_omega_e : DataTypeConversion  OutDataTypeStr=FOC_Fixed_Config.Types.Omega  RndMeth=Convergent
  Encode_theta_e : DataTypeConversion  OutDataTypeStr=FOC_Fixed_Config.Types.Angle  RndMeth=Convergent
  FOC_Model : ModelReference  ModelNameDialog=PMLSM_FOC_FixedPoint  SimulationMode=Normal  ModelReferenceVersion=1.26
  duty_u_cmd : Outport
  duty_v_cmd : Outport  Port=2
  duty_w_cmd : Outport  Port=3
  wires:
  ia/1 -> Encode_ia/1
  ib/1 -> Encode_ib/1
  ic/1 -> Encode_ic/1
  theta_e/1 -> Encode_theta_e/1
  omega_e/1 -> Encode_omega_e/1
  Vdc_V/1 -> Encode_Vdc_V/1
  iq_ref/1 -> Encode_iq_ref/1
  id_ref/1 -> Encode_id_ref/1
  PI_Reset_EN/1 -> Encode_PI_Reset_EN/1
  Encode_ia/1 -> FOC_Model/1
  Encode_theta_e/1 -> FOC_Model/4
  Encode_ic/1 -> FOC_Model/3
  Encode_ib/1 -> FOC_Model/2
  Encode_PI_Reset_EN/1 -> FOC_Model/8
  Encode_id_ref/1 -> FOC_Model/7
  Encode_iq_ref/1 -> FOC_Model/6
  Encode_omega_e/1 -> FOC_Model/5
  Encode_Vdc_V/1 -> FOC_Model/9
  FOC_Model/1 -> Decode_Duty1/1
  FOC_Model/2 -> Decode_Duty2/1
  FOC_Model/3 -> Decode_Duty3/1
  Decode_Duty3/1 -> duty_w_cmd/1
  Decode_Duty2/1 -> duty_v_cmd/1
  Decode_Duty1/1 -> duty_u_cmd/1

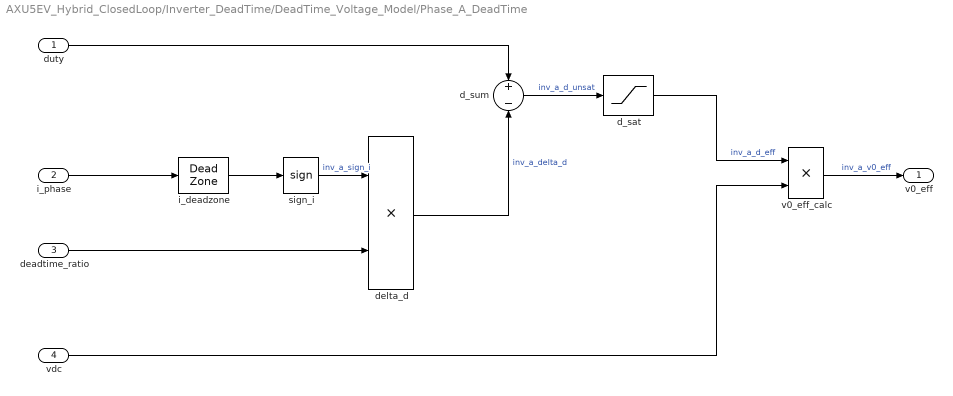
== system AXU5EV_Hybrid_ClosedLoop/Inverter_DeadTime/DeadTime_Voltage_Model/Phase_A_DeadTime ==
  duty : Inport
  i_phase : Inport  Port=2
  deadtime_ratio : Inport  Port=3
  vdc : Inport  Port=4
  d_sat : Saturate  UpperLimit=1  LowerLimit=0
  d_sum : Sum  Inputs=+-
  delta_d : Product  Inputs=**
  i_deadzone : DeadZone  LowerValue=-PMLSM_deadtime_current_eps_A  UpperValue=PMLSM_deadtime_current_eps_A
  sign_i : Signum
  v0_eff_calc : Product
  v0_eff : Outport
  wires:
  v0_eff_calc/1 -> v0_eff/1  "inv_a_v0_eff"
  vdc/1 -> v0_eff_calc/2
  d_sat/1 -> v0_eff_calc/1  "inv_a_d_eff"
  i_phase/1 -> i_deadzone/1
  i_deadzone/1 -> sign_i/1
  sign_i/1 -> delta_d/1  "inv_a_sign_i"
  deadtime_ratio/1 -> delta_d/2
  delta_d/1 -> d_sum/2  "inv_a_delta_d"
  d_sum/1 -> d_sat/1  "inv_a_d_unsat"
  duty/1 -> d_sum/1

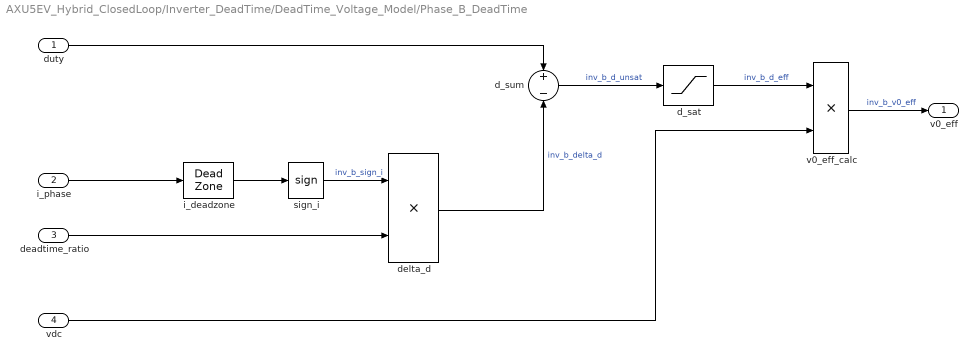
== system AXU5EV_Hybrid_ClosedLoop/Inverter_DeadTime/DeadTime_Voltage_Model/Phase_B_DeadTime ==
  duty : Inport
  i_phase : Inport  Port=2
  deadtime_ratio : Inport  Port=3
  vdc : Inport  Port=4
  d_sat : Saturate  UpperLimit=1  LowerLimit=0
  d_sum : Sum  Inputs=+-
  delta_d : Product  Inputs=**
  i_deadzone : DeadZone  LowerValue=-PMLSM_deadtime_current_eps_A  UpperValue=PMLSM_deadtime_current_eps_A
  sign_i : Signum
  v0_eff_calc : Product
  v0_eff : Outport
  wires:
  v0_eff_calc/1 -> v0_eff/1  "inv_b_v0_eff"
  vdc/1 -> v0_eff_calc/2
  d_sat/1 -> v0_eff_calc/1  "inv_b_d_eff"
  i_phase/1 -> i_deadzone/1
  i_deadzone/1 -> sign_i/1
  sign_i/1 -> delta_d/1  "inv_b_sign_i"
  deadtime_ratio/1 -> delta_d/2
  delta_d/1 -> d_sum/2  "inv_b_delta_d"
  d_sum/1 -> d_sat/1  "inv_b_d_unsat"
  duty/1 -> d_sum/1

== system AXU5EV_Hybrid_ClosedLoop/Inverter_DeadTime/DeadTime_Voltage_Model/Phase_C_DeadTime ==
  duty : Inport
  i_phase : Inport  Port=2
  deadtime_ratio : Inport  Port=3
  vdc : Inport  Port=4
  d_sat : Saturate  UpperLimit=1  LowerLimit=0
  d_sum : Sum  Inputs=+-
  delta_d : Product  Inputs=**
  i_deadzone : DeadZone  LowerValue=-PMLSM_deadtime_current_eps_A  UpperValue=PMLSM_deadtime_current_eps_A
  sign_i : Signum
  v0_eff_calc : Product
  v0_eff : Outport
  wires:
  v0_eff_calc/1 -> v0_eff/1  "inv_c_v0_eff"
  vdc/1 -> v0_eff_calc/2
  d_sat/1 -> v0_eff_calc/1  "inv_c_d_eff"
  i_phase/1 -> i_deadzone/1
  i_deadzone/1 -> sign_i/1
  sign_i/1 -> delta_d/1  "inv_c_sign_i"
  deadtime_ratio/1 -> delta_d/2
  delta_d/1 -> d_sum/2  "inv_c_delta_d"
  d_sum/1 -> d_sat/1  "inv_c_d_unsat"
  duty/1 -> d_sum/1

== matlab function AXU5EV_Hybrid_ClosedLoop/Command_Receipt/Receipt_Fields ==
  data: snapshot input; live output; commit input; receipt output
function [live,receipt] = fcn(snapshot,commit)
% 只读同次100 us输入/提交；不参与Ready判断或控制。
live=[snapshot(11);commit(31);commit(25)];
% 接收软件时间、Host状态、接受数、拒绝数、段号、接受目标mm。
receipt=[commit(35);commit(27);commit(32);commit(33);commit(34);commit(24)];
end
